simulink model "ASPA4"  (R2025b)
settings: Solver=VariableStepAuto  StartTime=0.0  StopTime=1  RelTol=1e-3
libraries: dspmlti4 x4, dspfdesign x3, dspstat3 x3, dspadpt3 x2, dspsrcs4 x1
settings Model: Creator=vishr  LastModifiedBy=vishr

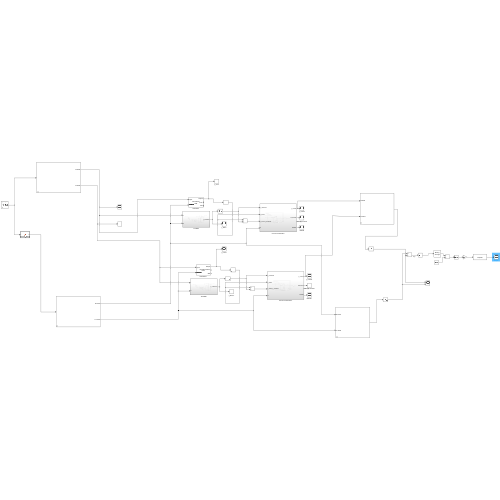
[thumbnail: Simulink's stored preview of the top-level diagram]
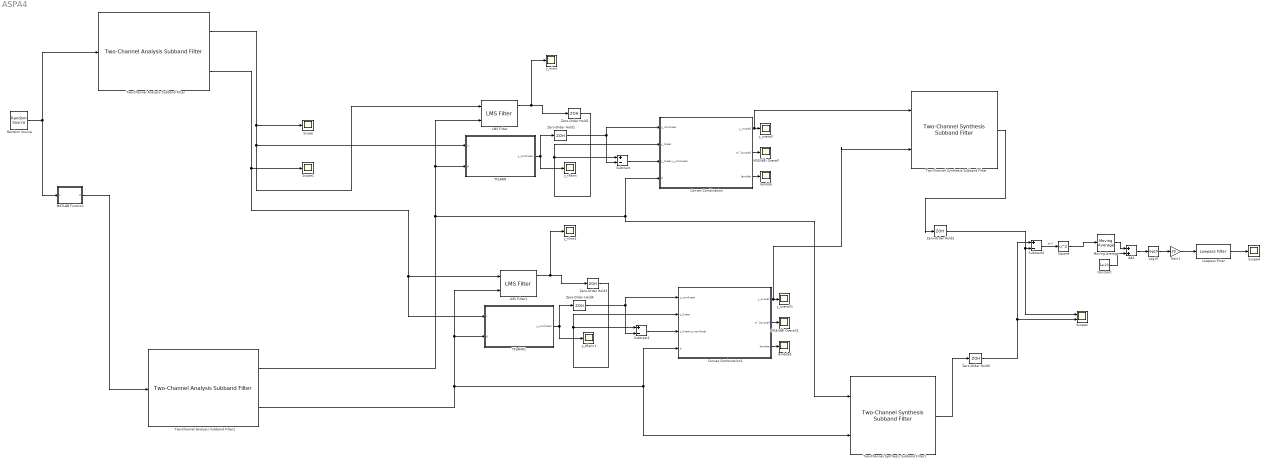
== system ASPA4 ==
  Add : Sum
  Constant : Constant  Value=1e-10
  Convex Combination : Subsystem
  Convex Combination1 : Subsystem
  Gain1 : Gain  Gain=20
  LMS Filter : dspadpt3/LMS Filter  Algo=Normalized LMS  L=10  stepflag=Dialog  mu=0.1  leakage=1.0  ic=0  Adapt=off  resetflag=None  weights=on  addnparflag=off  roundingMode=Floor  overflowMode=off  secondCoeffMode=Binary point scaling  secondCoeffWordLength=2  secondCoeffFracLength=15  prodOutput2Mode=Binary point scaling  prodOutput2FracLength=20  prodOutput3Mode=Binary point scaling  prodOutput3FracLength=20  prodOutput4Mode=Binary point scaling  prodOutput4FracLength=20  quotientMode=Binary point scaling  quotientFracLength=20  accum2Mode=Binary point scaling  accum2FracLength=20
      settings: LibrarySourceBlock=dsphdlsupportfiltering/LMS Filter
  LMS Filter1 : dspadpt3/LMS Filter  Algo=Normalized LMS  L=10  stepflag=Dialog  mu=0.1  leakage=1.0  ic=0  Adapt=off  resetflag=None  weights=on  addnparflag=off  roundingMode=Floor  overflowMode=off  secondCoeffMode=Binary point scaling  secondCoeffWordLength=2  secondCoeffFracLength=15  prodOutput2Mode=Binary point scaling  prodOutput2FracLength=20  prodOutput3Mode=Binary point scaling  prodOutput3FracLength=20  prodOutput4Mode=Binary point scaling  prodOutput4FracLength=20  quotientMode=Binary point scaling  quotientFracLength=20  accum2Mode=Binary point scaling  accum2FracLength=20
      settings: LibrarySourceBlock=dsphdlsupportfiltering/LMS Filter
  Log10 : Math  Operator=log10
  Lowpass Filter : dspfdesign/Lowpass Filter  FilterType=FIR  DesignForMinimumOrder=on  FilterOrder=50  PassbandFrequency=0.001  StopbandFrequency=0.03  PassbandRipple=0.1  StopbandAttenuation=80  SampleRateMode=Use normalized frequency (0 to 1)  SampleRate=44100  SimulateUsing=Interpreted execution  roundingMode=Floor  coeffsDataTypeStr=fixdt(1,16)
  MATLAB Function : MATLAB Function  TreatAsAtomicUnit=on
  MSE(dB) Overall : Scope
      settings: ActiveDisplayYMinimum=-39.306917327658191  ActiveDisplayYMaximum=4.3607467233555814  DataLoggingVariableName=ScopeData8
  MSE(dB) Overall1 : Scope
      settings: ActiveDisplayYMinimum=-41.5489552301683  ActiveDisplayYMaximum=4.6098620458567057  DataLoggingVariableName=ScopeData2
  Moving Average : dspstat3/Moving Average  Method=Sliding window  ForgettingFactorPort=off  SpecifyWindowLength=on  WindowLength=4  OverlapLength=3  AllowArbitraryInputLength=off  ForgettingFactor=0.9  SimulateUsing=Interpreted execution
  Random Source : dspsrcs4/Random Source  SrcType=Gaussian  MinVal=0  MaxVal=1  MeanVal=0  VarVal=1  RepMode=Specify seed  rawSeed=1  IsInherit=off  SampTime=1e-4  SampFrame=1  OutComplex=Real  DataType=double  SimulateUsing=Interpreted execution
  Scope : Scope
      settings: ActiveDisplayYMinimum=-3.5548608937660848  ActiveDisplayYMaximum=3.6041755939414184  DataLoggingVariableName=ScopeData10
  Scope1 : Scope
      settings: ActiveDisplayYMinimum=-3.5818003621766747  ActiveDisplayYMaximum=3.6930911677490457  DataLoggingVariableName=ScopeData11
  Scope2 : Scope  NumInputPorts=2
      settings: ActiveDisplayYMinimum=-2.1098463486901959  ActiveDisplayYMaximum=2.0164123844325865  DataLoggingVariableName=ScopeData12
  Scope4 : Scope
      settings: ActiveDisplayYMinimum=-50  ActiveDisplayYMaximum=20  DataLoggingVariableName=ScopeData14
  Square : Math  Operator=square
  Subtract : Sum  Inputs=+-
  Subtract1 : Sum  Inputs=+-
  Subtract2 : Sum  Inputs=+-
  TFLANN : Subsystem
  TFLANN1 : Subsystem
  Two-Channel Analysis Subband Filter : dspmlti4/Two-Channel Analysis Subband Filter  lpf=[0.0094, -0.0707, 0.0694, 0.4900, 0.4900, 0.0694, -0.0707, 0.0094]  hpf=[0.0094, 0.0707, 0.0694, -0.4900, 0.4900, -0.0694, -0.0707, -0.0094]  InputProcessing=Columns as channels (frame based)  framing=Allow multirate processing  AllowArbitraryInputLength=off  roundingMode=Floor  overflowMode=off  firstCoeffDataTypeStr=Inherit: Same word length as input  firstCoeffMin=[]  firstCoeffMax=[]  firstCoeffLastDataTypeStr=Inherit: Same word length as input  outputDataTypeStr=Inherit: Same as accumulator  outputMin=[]  outputMax=[]  outputLastDataTypeStr=Inherit: Same as accumulator
  Two-Channel Analysis Subband Filter1 : dspmlti4/Two-Channel Analysis Subband Filter  lpf=[0.0094, -0.0707, 0.0694, 0.4900, 0.4900, 0.0694, -0.0707, 0.0094]  hpf=[0.0094, 0.0707, 0.0694, -0.4900, 0.4900, -0.0694, -0.0707, -0.0094]  InputProcessing=Columns as channels (frame based)  framing=Allow multirate processing  AllowArbitraryInputLength=off  roundingMode=Floor  overflowMode=off  firstCoeffDataTypeStr=Inherit: Same word length as input  firstCoeffMin=[]  firstCoeffMax=[]  firstCoeffLastDataTypeStr=Inherit: Same word length as input  outputDataTypeStr=Inherit: Same as accumulator  outputMin=[]  outputMax=[]  outputLastDataTypeStr=Inherit: Same as accumulator
  Two-Channel Synthesis Subband Filter : dspmlti4/Two-Channel Synthesis Subband Filter  lpf=[0.0094, -0.0707, 0.0694, 0.4900, 0.4900, 0.0694, -0.0707, 0.0094]  hpf=[0.0094, 0.0707, 0.0694, -0.4900, 0.4900, -0.0694, -0.0707, -0.0094]  InputProcessing=Columns as channels (frame based)  framing=Allow multirate processing  roundingMode=Floor  overflowMode=off  firstCoeffDataTypeStr=Inherit: Same word length as input  firstCoeffMin=[]  firstCoeffMax=[]  firstCoeffLastDataTypeStr=Inherit: Same word length as input  outputDataTypeStr=Inherit: Same as accumulator  outputMin=[]  outputMax=[]  outputLastDataTypeStr=Inherit: Same as accumulator
  Two-Channel Synthesis Subband Filter1 : dspmlti4/Two-Channel Synthesis Subband Filter  lpf=[0.0094, -0.0707, 0.0694, 0.4900, 0.4900, 0.0694, -0.0707, 0.0094]  hpf=[0.0094, 0.0707, 0.0694, -0.4900, 0.4900, -0.0694, -0.0707, -0.0094]  InputProcessing=Columns as channels (frame based)  framing=Allow multirate processing  roundingMode=Floor  overflowMode=off  firstCoeffDataTypeStr=Inherit: Same word length as input  firstCoeffMin=[]  firstCoeffMax=[]  firstCoeffLastDataTypeStr=Inherit: Same word length as input  outputDataTypeStr=Inherit: Same as accumulator  outputMin=[]  outputMax=[]  outputLastDataTypeStr=Inherit: Same as accumulator
  Zero-Order Hold{1..6} (6 alike) : ZeroOrderHold  SampleTime=1e-4
  lambda : Scope
      settings: ActiveDisplayYMinimum=-1  ActiveDisplayYMaximum=1  DataLoggingVariableName=ScopeData9
  lambda1 : Scope
      settings: ActiveDisplayYMinimum=-1  ActiveDisplayYMaximum=1  DataLoggingVariableName=ScopeData3
  y_nlms : Scope
  y_nlms1 : Scope
      settings: DataLoggingVariableName=ScopeData4
  y_overall : Scope
      settings: ActiveDisplayYMinimum=-3.93121235585972  ActiveDisplayYMaximum=4.0932209788377252  DataLoggingVariableName=ScopeData5
  y_overall1 : Scope
      settings: ActiveDisplayYMinimum=-3.93121235585972  ActiveDisplayYMaximum=4.0932209788377252  DataLoggingVariableName=ScopeData6
  y_tflann : Scope
      settings: ActiveDisplayYMinimum=-2.0302293992486709  ActiveDisplayYMaximum=2.2383486881688421
  y_tflann1 : Scope
      settings: ActiveDisplayYMinimum=-2.0302293992486709  ActiveDisplayYMaximum=2.2383486881688421  DataLoggingVariableName=ScopeData7
  wires:
  Convex Combination/3(lambda) -> lambda/1
  LMS Filter/1 -> y_nlms/1, Zero-Order Hold1/1
  Two-Channel Analysis Subband Filter1/1 -> LMS Filter/2, TFLANN/2(d), Convex Combination/4(d), Two-Channel Synthesis Subband Filter1/1
  Zero-Order Hold1/1 -> Subtract/1, Convex Combination/2(y_linear)
  Convex Combination/1(y_overall) -> Two-Channel Synthesis Subband Filter/1, y_overall/1
  Zero-Order Hold2/1 -> Subtract/2, Convex Combination/1(y_nonlinear)
  TFLANN/1(y_nonlinear) -> y_tflann/1, Zero-Order Hold2/1
  Random Source/1 -> MATLAB Function/1(x), Two-Channel Analysis Subband Filter/1
  Convex Combination/2(e^2overall) -> MSE(dB) Overall/1
  Subtract/1 -> Convex Combination/3(y_linear-y_nonlinear)
  Subtract1/1 -> Convex Combination1/3(y_linear-y_nonlinear)
  Convex Combination1/3(lambda) -> lambda1/1
  LMS Filter1/1 -> y_nlms1/1, Zero-Order Hold3/1
  Two-Channel Analysis Subband Filter/2 -> TFLANN1/1(x), LMS Filter1/1, Scope1/1
  Zero-Order Hold4/1 -> Subtract1/2, Convex Combination1/1(y_nonlinear)
  Zero-Order Hold3/1 -> Subtract1/1, Convex Combination1/2(y_linear)
  Convex Combination1/2(e^2overall) -> MSE(dB) Overall1/1
  TFLANN1/1(y_nonlinear) -> y_tflann1/1, Zero-Order Hold4/1
  Two-Channel Analysis Subband Filter1/2 -> LMS Filter1/2, TFLANN1/2(d), Convex Combination1/4(d), Two-Channel Synthesis Subband Filter1/2
  Convex Combination1/1(y_overall) -> Two-Channel Synthesis Subband Filter/2, y_overall1/1
  Zero-Order Hold6/1 -> Subtract2/1, Scope2/2
  Zero-Order Hold5/1 -> Scope2/1, Subtract2/2
  Subtract2/1 -> Square/1  "e(n)"
  Gain1/1 -> Lowpass Filter/1
  Square/1 -> Moving Average/1
  Log10/1 -> Gain1/1
  Moving Average/1 -> Add/1
  Add/1 -> Log10/1
  Constant/1 -> Add/2
  Two-Channel Synthesis Subband Filter/1 -> Zero-Order Hold5/1
  MATLAB Function/1(d) -> Two-Channel Analysis Subband Filter1/1
  Lowpass Filter/1 -> Scope4/1
  Two-Channel Synthesis Subband Filter1/1 -> Zero-Order Hold6/1
  Two-Channel Analysis Subband Filter/1 -> LMS Filter/1, TFLANN/1(x), Scope/1

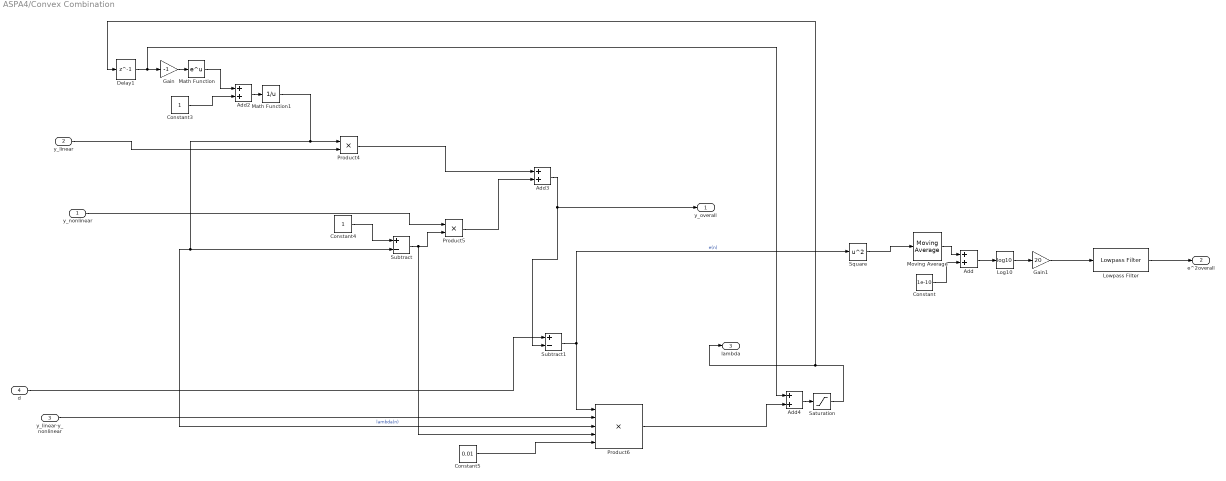
== system ASPA4/Convex Combination ==
  y_nonlinear : Inport
  y_linear : Inport  Port=2
  y_linear-y_nonlinear : Inport  Port=3
  d : Inport  Port=4
  Add{,2..4} (4 alike) : Sum
  Constant : Constant  Value=1e-10
  Constant3 : Constant
  Constant4 : Constant
  Constant5 : Constant  Value=0.01
  Delay1 : Delay  DelayLength=1  InputProcessing=Columns as channels (frame based)
  Gain : Gain  Gain=-1
  Gain1 : Gain  Gain=20
  Log10 : Math  Operator=log10
  Lowpass Filter : dspfdesign/Lowpass Filter  FilterType=FIR  DesignForMinimumOrder=on  FilterOrder=50  PassbandFrequency=0.001  StopbandFrequency=0.03  PassbandRipple=0.1  StopbandAttenuation=80  SampleRateMode=Use normalized frequency (0 to 1)  SampleRate=44100  SimulateUsing=Interpreted execution  roundingMode=Floor  coeffsDataTypeStr=fixdt(1,16)
  Math Function : Math
  Math Function1 : Math  Operator=reciprocal
  Moving Average : dspstat3/Moving Average  Method=Sliding window  ForgettingFactorPort=off  SpecifyWindowLength=on  WindowLength=4  OverlapLength=3  AllowArbitraryInputLength=off  ForgettingFactor=0.9  SimulateUsing=Interpreted execution
  Product4 : Product
  Product5 : Product
  Product6 : Product  Inputs=5
  Saturation : Saturate  UpperLimit=1  LowerLimit=0
  Square : Math  Operator=square
  Subtract : Sum  Inputs=+-
  Subtract1 : Sum  Inputs=+-
  y_overall : Outport
  e^2overall : Outport  Port=2
  lambda : Outport  Port=3
  wires:
  Add2/1 -> Math Function1/1
  Math Function/1 -> Add2/1
  y_nonlinear/1 -> Product5/1
  Subtract1/1 -> Square/1, Product6/1  "e(n)"
  Product6/1 -> Add4/2
  Math Function1/1 -> Product4/1, Product6/3, Subtract/2  "lambda(n)"
  Subtract/1 -> Product6/4, Product5/2
  y_linear/1 -> Product4/2
  Saturation/1 -> lambda/1, Delay1/1
  Constant3/1 -> Add2/2
  Constant5/1 -> Product6/5
  Add3/1 -> y_overall/1, Subtract1/2
  Gain/1 -> Math Function/1
  Constant4/1 -> Subtract/1
  Product5/1 -> Add3/2
  Delay1/1 -> Add4/1, Gain/1
  Product4/1 -> Add3/1
  d/1 -> Subtract1/1
  y_linear-y_nonlinear/1 -> Product6/2
  Add4/1 -> Saturation/1
  Square/1 -> Moving Average/1
  Moving Average/1 -> Add/1
  Constant/1 -> Add/2
  Add/1 -> Log10/1
  Log10/1 -> Gain1/1
  Gain1/1 -> Lowpass Filter/1
  Lowpass Filter/1 -> e^2overall/1

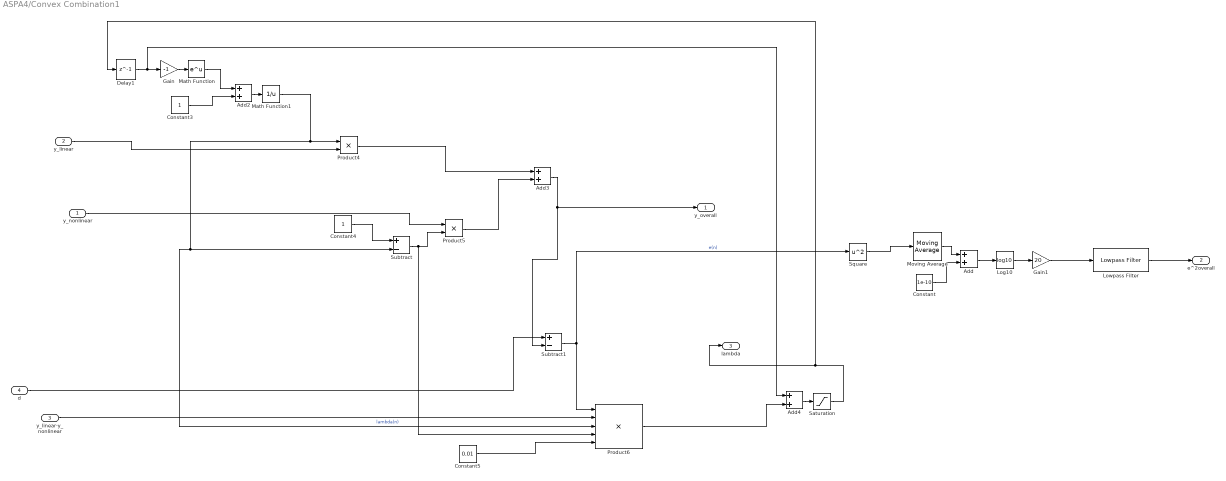
== system ASPA4/Convex Combination1 ==
  y_nonlinear : Inport
  y_linear : Inport  Port=2
  y_linear-y_nonlinear : Inport  Port=3
  d : Inport  Port=4
  Add{,2..4} (4 alike) : Sum
  Constant : Constant  Value=1e-10
  Constant3 : Constant
  Constant4 : Constant
  Constant5 : Constant  Value=0.01
  Delay1 : Delay  DelayLength=1  InputProcessing=Columns as channels (frame based)
  Gain : Gain  Gain=-1
  Gain1 : Gain  Gain=20
  Log10 : Math  Operator=log10
  Lowpass Filter : dspfdesign/Lowpass Filter  FilterType=FIR  DesignForMinimumOrder=on  FilterOrder=50  PassbandFrequency=0.001  StopbandFrequency=0.03  PassbandRipple=0.1  StopbandAttenuation=80  SampleRateMode=Use normalized frequency (0 to 1)  SampleRate=44100  SimulateUsing=Interpreted execution  roundingMode=Floor  coeffsDataTypeStr=fixdt(1,16)
  Math Function : Math
  Math Function1 : Math  Operator=reciprocal
  Moving Average : dspstat3/Moving Average  Method=Sliding window  ForgettingFactorPort=off  SpecifyWindowLength=on  WindowLength=4  OverlapLength=3  AllowArbitraryInputLength=off  ForgettingFactor=0.9  SimulateUsing=Interpreted execution
  Product4 : Product
  Product5 : Product
  Product6 : Product  Inputs=5
  Saturation : Saturate  UpperLimit=1  LowerLimit=0
  Square : Math  Operator=square
  Subtract : Sum  Inputs=+-
  Subtract1 : Sum  Inputs=+-
  y_overall : Outport
  e^2overall : Outport  Port=2
  lambda : Outport  Port=3
  wires:
  Add2/1 -> Math Function1/1
  Math Function/1 -> Add2/1
  y_nonlinear/1 -> Product5/1
  Subtract1/1 -> Square/1, Product6/1  "e(n)"
  Product6/1 -> Add4/2
  Math Function1/1 -> Product4/1, Product6/3, Subtract/2  "lambda(n)"
  Subtract/1 -> Product6/4, Product5/2
  y_linear/1 -> Product4/2
  Saturation/1 -> lambda/1, Delay1/1
  Constant3/1 -> Add2/2
  Constant5/1 -> Product6/5
  Add3/1 -> y_overall/1, Subtract1/2
  Gain/1 -> Math Function/1
  Constant4/1 -> Subtract/1
  Product5/1 -> Add3/2
  Delay1/1 -> Add4/1, Gain/1
  Product4/1 -> Add3/1
  d/1 -> Subtract1/1
  y_linear-y_nonlinear/1 -> Product6/2
  Add4/1 -> Saturation/1
  Square/1 -> Moving Average/1
  Moving Average/1 -> Add/1
  Constant/1 -> Add/2
  Add/1 -> Log10/1
  Log10/1 -> Gain1/1
  Gain1/1 -> Lowpass Filter/1
  Lowpass Filter/1 -> e^2overall/1

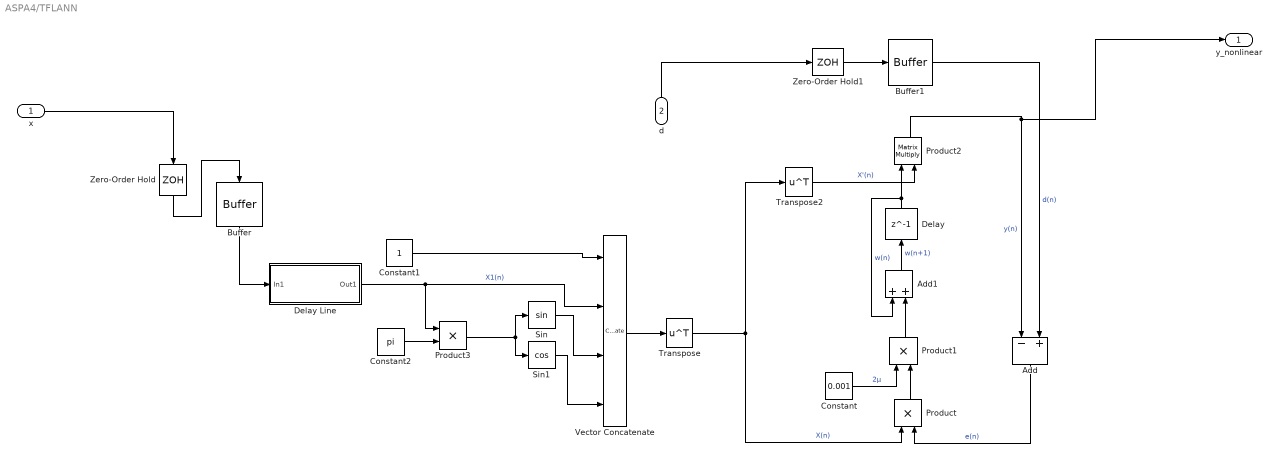
== system ASPA4/TFLANN ==
  x : Inport
  d : Inport  Port=2
  Add : Sum  Inputs=-+
  Add1 : Sum
  Buffer : Buffer  N=1  OutputFrames=off
  Buffer1 : Buffer  N=1  OutputFrames=off
  Constant : Constant  Value=0.001
  Constant1 : Constant
  Constant2 : Constant  Value=pi
  Delay : Delay  DelayLength=1  InputProcessing=Columns as channels (frame based)
  Delay Line : Subsystem
  Product : Product
  Product1 : Product
  Product2 : Product  Multiplication=Matrix(*)
  Product3 : Product
  Sin : Trigonometry
  Sin1 : Trigonometry  Operator=cos
  Transpose : Math  Operator=transpose
  Transpose2 : Math  Operator=transpose
  Vector Concatenate : Concatenate  NumInputs=4
  Zero-Order Hold : ZeroOrderHold  SampleTime=1/(6e3)
  Zero-Order Hold1 : ZeroOrderHold  SampleTime=1/(6e3)
  y_nonlinear : Outport
  wires:
  Transpose2/1 -> Product2/2  "X'(n)"
  Add/1 -> Product/2  "e(n)"
  Delay Line/1(Out1) -> Vector Concatenate/2, Product3/1  "X1(n)"
  Sin1/1 -> Vector Concatenate/4
  Product1/1 -> Add1/2
  Product/1 -> Product1/2
  Delay/1 -> Add1/1, Product2/1  "w(n)"
  Sin/1 -> Vector Concatenate/3
  Vector Concatenate/1 -> Transpose/1
  Constant/1 -> Product1/1  "2μ"
  Add1/1 -> Delay/1  "w(n+1)"
  Product2/1 -> Add/1, y_nonlinear/1  "y(n)"
  Transpose/1 -> Transpose2/1, Product/1  "X(n)"
  Zero-Order Hold/1 -> Buffer/1
  Constant2/1 -> Product3/2
  Buffer1/1 -> Add/2  "d(n)"
  Product3/1 -> Sin/1, Sin1/1
  Constant1/1 -> Vector Concatenate/1
  Buffer/1 -> Delay Line/1(In1)
  Zero-Order Hold1/1 -> Buffer1/1
  x/1 -> Zero-Order Hold/1
  d/1 -> Zero-Order Hold1/1

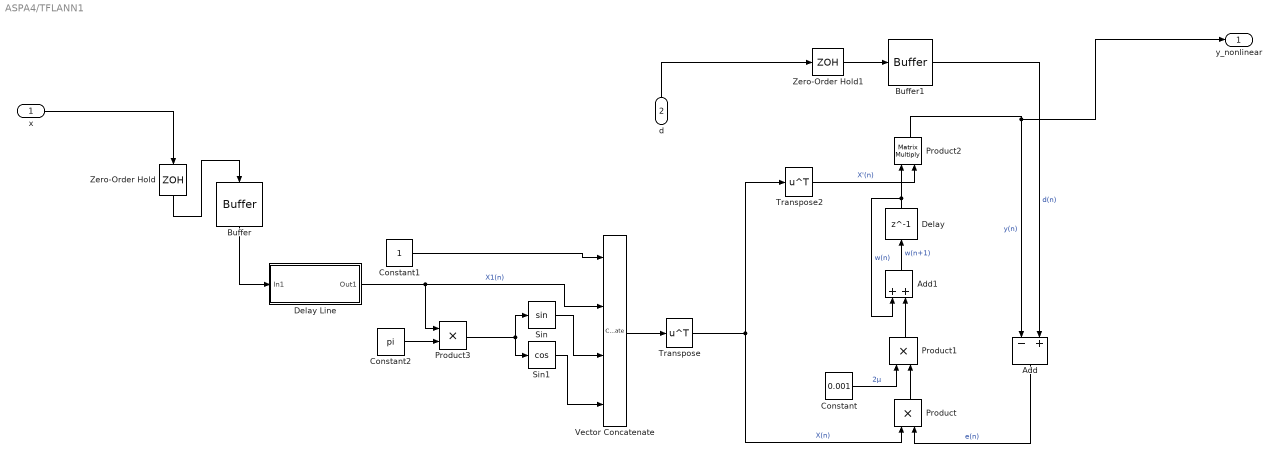
== system ASPA4/TFLANN1 ==
  x : Inport
  d : Inport  Port=2
  Add : Sum  Inputs=-+
  Add1 : Sum
  Buffer : Buffer  N=1  OutputFrames=off
  Buffer1 : Buffer  N=1  OutputFrames=off
  Constant : Constant  Value=0.001
  Constant1 : Constant
  Constant2 : Constant  Value=pi
  Delay : Delay  DelayLength=1  InputProcessing=Columns as channels (frame based)
  Delay Line : Subsystem
  Product : Product
  Product1 : Product
  Product2 : Product  Multiplication=Matrix(*)
  Product3 : Product
  Sin : Trigonometry
  Sin1 : Trigonometry  Operator=cos
  Transpose : Math  Operator=transpose
  Transpose2 : Math  Operator=transpose
  Vector Concatenate : Concatenate  NumInputs=4
  Zero-Order Hold : ZeroOrderHold  SampleTime=1/(6e3)
  Zero-Order Hold1 : ZeroOrderHold  SampleTime=1/(6e3)
  y_nonlinear : Outport
  wires:
  Transpose2/1 -> Product2/2  "X'(n)"
  Add/1 -> Product/2  "e(n)"
  Delay Line/1(Out1) -> Vector Concatenate/2, Product3/1  "X1(n)"
  Sin1/1 -> Vector Concatenate/4
  Product1/1 -> Add1/2
  Product/1 -> Product1/2
  Delay/1 -> Add1/1, Product2/1  "w(n)"
  Sin/1 -> Vector Concatenate/3
  Vector Concatenate/1 -> Transpose/1
  Constant/1 -> Product1/1  "2μ"
  Add1/1 -> Delay/1  "w(n+1)"
  Product2/1 -> Add/1, y_nonlinear/1  "y(n)"
  Transpose/1 -> Transpose2/1, Product/1  "X(n)"
  Zero-Order Hold/1 -> Buffer/1
  Constant2/1 -> Product3/2
  Buffer1/1 -> Add/2  "d(n)"
  Product3/1 -> Sin/1, Sin1/1
  Constant1/1 -> Vector Concatenate/1
  Buffer/1 -> Delay Line/1(In1)
  Zero-Order Hold1/1 -> Buffer1/1
  x/1 -> Zero-Order Hold/1
  d/1 -> Zero-Order Hold1/1

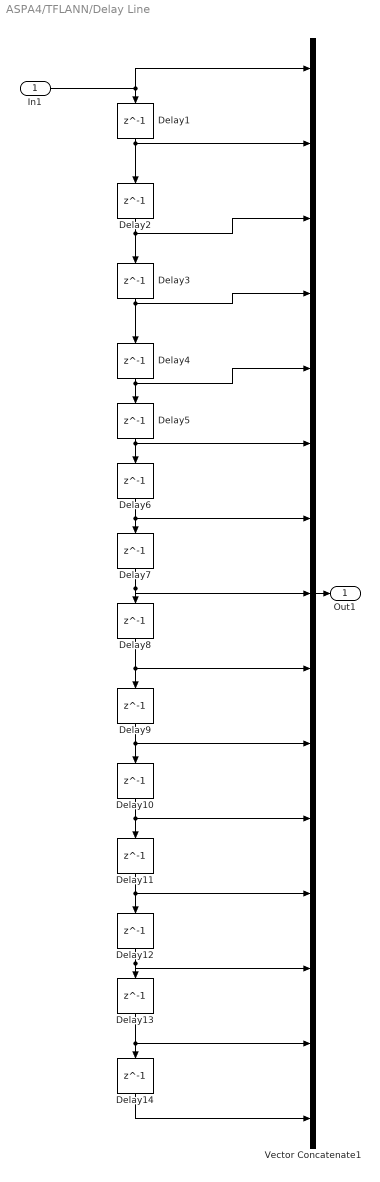
== system ASPA4/TFLANN/Delay Line ==
  In1 : Inport
  Delay{1..14} (14 alike) : Delay  DelayLength=1  InputProcessing=Columns as channels (frame based)
  Vector Concatenate1 : Concatenate  NumInputs=15
  Out1 : Outport
  wires:
  Delay14/1 -> Vector Concatenate1/15
  Delay5/1 -> Delay6/1, Vector Concatenate1/6
  Delay6/1 -> Delay7/1, Vector Concatenate1/7
  Delay3/1 -> Delay4/1, Vector Concatenate1/4
  Delay8/1 -> Delay9/1, Vector Concatenate1/9
  Delay12/1 -> Vector Concatenate1/13, Delay13/1
  In1/1 -> Delay1/1, Vector Concatenate1/1
  Delay13/1 -> Vector Concatenate1/14, Delay14/1
  Delay7/1 -> Delay8/1, Vector Concatenate1/8
  Delay11/1 -> Vector Concatenate1/12, Delay12/1
  Delay2/1 -> Delay3/1, Vector Concatenate1/3
  Delay9/1 -> Delay10/1, Vector Concatenate1/10
  Delay4/1 -> Vector Concatenate1/5, Delay5/1
  Delay1/1 -> Delay2/1, Vector Concatenate1/2
  Delay10/1 -> Delay11/1, Vector Concatenate1/11
  Vector Concatenate1/1 -> Out1/1

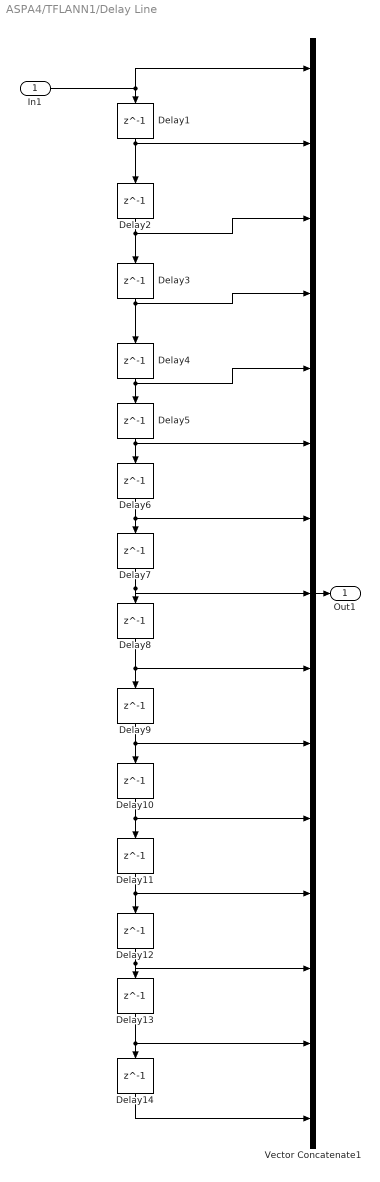
== system ASPA4/TFLANN1/Delay Line ==
  In1 : Inport
  Delay{1..14} (14 alike) : Delay  DelayLength=1  InputProcessing=Columns as channels (frame based)
  Vector Concatenate1 : Concatenate  NumInputs=15
  Out1 : Outport
  wires:
  Delay14/1 -> Vector Concatenate1/15
  Delay5/1 -> Delay6/1, Vector Concatenate1/6
  Delay6/1 -> Delay7/1, Vector Concatenate1/7
  Delay3/1 -> Delay4/1, Vector Concatenate1/4
  Delay8/1 -> Delay9/1, Vector Concatenate1/9
  Delay12/1 -> Vector Concatenate1/13, Delay13/1
  In1/1 -> Delay1/1, Vector Concatenate1/1
  Delay13/1 -> Vector Concatenate1/14, Delay14/1
  Delay7/1 -> Delay8/1, Vector Concatenate1/8
  Delay11/1 -> Vector Concatenate1/12, Delay12/1
  Delay2/1 -> Delay3/1, Vector Concatenate1/3
  Delay9/1 -> Delay10/1, Vector Concatenate1/10
  Delay4/1 -> Vector Concatenate1/5, Delay5/1
  Delay1/1 -> Delay2/1, Vector Concatenate1/2
  Delay10/1 -> Delay11/1, Vector Concatenate1/11
  Vector Concatenate1/1 -> Out1/1

== matlab function ASPA4/MATLAB Function ==
  data: x input; d output
function d = unknown_system(x)
    persistent delay_line n;
    
    if isempty(delay_line)
        delay_line = zeros(5, 1);
        n = 0;
    end

    n = n + 1;

    delay_line = [x; delay_line(1:end-1)];
    w_true = [0.8; -0.4; 0.2; -0.1; 0.05];
    
    y_linear = w_true' * delay_line;

    y_clean = y_linear + 0.2 * sin(pi*y_linear) - 0.1 * cos(pi*y_linear);
    noise = 0.0316 * randn();

    d = y_clean + noise;
end
